simulink model "springdamper_model"  (R2020a)
settings: Solver=ode45  StartTime=0.0  StopTime=4  MaxStep=0.0009  MinStep=0.0001  RelTol=1e-3
values from neighbouring files (symbols this model uses):
  C_W = 1000    [springdamper_data.m]
  H_PC = 0.1265    [springdamper_data.m]
  H_RC_FRONT = 0.0346    [springdamper_data.m]
  H_RC_REAR = 0.0779    [springdamper_data.m]
  K_S = 26300    [springdamper_data.m]
  K_W = 50000    [springdamper_data.m]
  PC_TO_FRONT_AXLE = 0.667    [springdamper_data.m]
  PC_TO_REAR_AXLE = WHEELBASE-0.667    (= 0.873)    [springdamper_data.m]
  PITCH_INERTIA_PC = PITCH_INERTIA + SUSP_MASS*PC_TO_SUSPCOG^2    (= 73.7412)    [springdamper_data.m]
  pull = pull15431543    [springdamper_data.m]
  push = push15431543    [springdamper_data.m]
  QUARTER_MASS = 13    [springdamper_data.m]
  RC_TO_WHEEL_FRONT = TRACK_FRONT/2    (= 0.6)    [springdamper_data.m]
  RC_TO_WHEEL_REAR = TRACK_REAR/2    (= 0.58)    [springdamper_data.m]
  ROLL_INERTIA_RC = ROLL_INERTIA + SUSP_MASS*((RC_TO_SUSPCOG_FRONT+RC_TO_SUSPCOG_REAR)/2)^2    (= 22.694437)    [springdamper_data.m]
  SUSP_MASS = 208    [springdamper_data.m]
  SUSPCOG = 0.283    [springdamper_data.m]
  vel = [0 12.5 25 50 75 100 125 150 175 200 225 250]    [springdamper_data.m]
  WHEELBASE = 1.54    [springdamper_data.m]
  YAW_INERTIA = 63    [springdamper_data.m]
undefined symbols (not defined in the file or in its folder): sigbuilder_block
libraries: simulink_extras x6, simulink x3
(part 1 of 2)
settings Model: Creator=pungorpeter  LastModifiedBy=pungorpeter

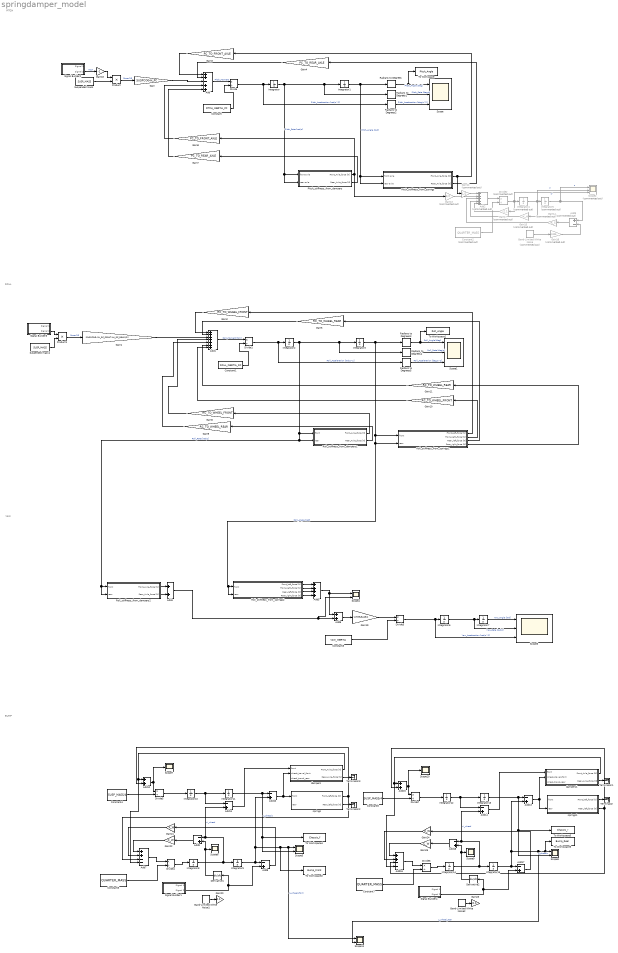
== system springdamper_model ==
  note: BUMP
  note: YAW
  note: ROLL
  note: PITCH
  Add : Sum  Inputs=++-++
  Add1 : Sum  Inputs=+++++++
  Add{8..11,13..14,17..18} (8 alike) : Sum  Inputs=-+
  Add{4,6,12,15} (4 alike) : Sum
  Add16 : Sum  Inputs=++--
  Add2 : Sum  Commented=on  Inputs=+++++
  Add3 : Sum  Commented=on  Inputs=+-
  Add5 : Sum  Inputs=++++
  Add7 : Sum  Inputs=++--
  Band-Limited White Noise : simulink/Sources/Band-Limited White Noise  Commented=on  Cov=[0.0005]  Ts=0.05  seed=[54341]
  Band-Limited White Noise1 : simulink/Sources/Band-Limited White Noise  Cov=[0.0005]  Ts=0.05  seed=[54341]
  Band-Limited White Noise2 : simulink/Sources/Band-Limited White Noise  Cov=[0.0005]  Ts=0.05  seed=[54341]
  Constant : Constant  Value=PITCH_INERTIA_PC
  Constant1 : Constant  Value=ROLL_INERTIA_RC
  Constant2 : Constant  Commented=on  Value=QUARTER_MASS
  Constant3 : Constant  Value=YAW_INERTIA
  Constant4 : Constant  Value=SUSP_MASS/4
  Constant5 : Constant  Value=QUARTER_MASS
  Constant6 : Constant  Value=SUSP_MASS/4
  Constant7 : Constant  Value=QUARTER_MASS
  Derivative1 : Derivative
  Derivative2 : Derivative
  Divide{,1,3..7} (7 alike) : Product  Inputs=*/
  Divide2 : Product  Commented=on  Inputs=*/
  Gain : Gain  Gain=SUSPCOG-H_PC
  Gain1 : Gain  Gain=(SUSPCOG-((H_RC_FRONT+H_RC_REAR)/2))
  Gain10 : Gain  Gain=RC_TO_WHEEL_FRONT
  Gain11 : Gain  Gain=RC_TO_WHEEL_REAR
  Gain12 : Gain  Commented=on  Gain=1/2
  Gain13 : Gain  Commented=on  Gain=1/2
  Gain14 : Gain  Commented=on  Gain=-K_S
  Gain15 : Gain  Commented=on  Gain=-K_W
  Gain16 : Gain  Commented=on  Gain=0.005
  Gain17 : Gain  Commented=on  Gain=-2.1
  Gain18 : Gain  Gain=-1
  Gain19 : Gain  Gain=WHEELBASE/2
  Gain2 : Gain  Gain=RC_TO_WHEEL_FRONT
  Gain20 : Gain  Gain=0.1
  Gain21 : Gain  Gain=K_W
  Gain22 : Gain  Gain=C_W
  Gain23 : Gain  Gain=0.1
  Gain24 : Gain  Gain=K_W
  Gain25 : Gain  Gain=C_W
  Gain3 : Gain  Gain=PC_TO_FRONT_AXLE
  Gain4 : Gain  Gain=PC_TO_REAR_AXLE
  Gain5 : Gain  Gain=RC_TO_WHEEL_REAR
  Gain6 : Gain  Gain=RC_TO_WHEEL_FRONT
  Gain7 : Gain  Gain=PC_TO_REAR_AXLE
  Gain8 : Gain  Gain=PC_TO_FRONT_AXLE
  Gain9 : Gain  Gain=RC_TO_WHEEL_REAR
  Integrator{,1..3,6..15} (14 alike) : Integrator
  Integrator4 : Integrator  Commented=on
  Integrator5 : Integrator  Commented=on
  Pitch_stiffness_from_dampers : Subsystem
  Pitch_stiffness_from_springs : Subsystem
  Product : Product
  Product1 : Product
  Radians to Degrees{,1..5} (6 alike) : simulink_extras/Transformations/Radians to Degrees
  Roll_stiffness_from_dampers1 : Subsystem
  Roll_stiffness_from_dampers2 : Subsystem
  Roll_stiffness_from_springs1 : Subsystem
  Roll_stiffness_from_springs2 : Subsystem
  Scope : Scope  NumInputPorts=3
  Scope1 : Scope  NumInputPorts=3
  Scope{6..7,9..10} (4 alike) : Scope
  Scope{4..5,8,11} (4 alike) : Scope  NumInputPorts=2
  Scope2 : Scope  Commented=on  NumInputPorts=3
  Scope3 : Scope  NumInputPorts=3
  Signal Builder1 : Subsystem  Tag=STV Subsys  LoadFcn=sigbuilder_block('load');  StartFcn=sigbuilder_block('start');  StopFcn=sigbuilder_block('stop');  ClipboardFcn=sigbuilder_block('clipboard');  mask(Sigbuilder block){tuvar=[0:10]}
      mask help: Simulink:masks:SigbuilderBlock_MD
      mask init:
      | if ~strcmp(get_param(bdroot(gcbh),'SimulationStatus'),'stopped') tuvar = sigbuilder_block('maskInit'); end
      settings: CopyFcn=sigbuilder_block('copy');  DeleteFcn=sigbuilder_block('delete');  ModelCloseFcn=sigbuilder_block('modelClose');  PreSaveFcn=sigbuilder_block('preSave');  PauseFcn=sigbuilder_block('pause');  ContinueFcn=sigbuilder_block('continue');  NameChangeFcn=sigbuilder_block('namechange');  OpenFcn=sigbuilder_block('open',[346.8 134.4 550.8 400.2 ]);  CloseFcn=sigbuilder_block('close');
      mask Display: plot(0, 0, 100, 100,[2, 2, 32, 32, 2], [68, 8, 8, 68, 68],[32, 2], [38, 38], [32, 19, 2],[53, 60, 44], [32, 17, 17, 2],[16, 16, 31, 31]);txt = getActiveGroup(gcbh);text(2, 100, txt,'verticalAlignment', 'top');
  Signal Builder2 : Subsystem  Tag=STV Subsys  LoadFcn=sigbuilder_block('load');  StartFcn=sigbuilder_block('start');  StopFcn=sigbuilder_block('stop');  ClipboardFcn=sigbuilder_block('clipboard');  mask(Sigbuilder block){tuvar=[0:10]}
      mask help: Simulink:masks:SigbuilderBlock_MD
      mask init:
      | if ~strcmp(get_param(bdroot(gcbh),'SimulationStatus'),'stopped') tuvar = sigbuilder_block('maskInit'); end
      settings: CopyFcn=sigbuilder_block('copy');  DeleteFcn=sigbuilder_block('delete');  ModelCloseFcn=sigbuilder_block('modelClose');  PreSaveFcn=sigbuilder_block('preSave');  PauseFcn=sigbuilder_block('pause');  ContinueFcn=sigbuilder_block('continue');  NameChangeFcn=sigbuilder_block('namechange');  OpenFcn=sigbuilder_block('open',[346.8 134.4 550.8 400.2 ]);  CloseFcn=sigbuilder_block('close');
      mask Display: plot(0, 0, 100, 100,[2, 2, 32, 32, 2], [68, 8, 8, 68, 68],[32, 2], [38, 38], [32, 19, 2],[53, 60, 44], [32, 17, 17, 2],[16, 16, 31, 31]);txt = getActiveGroup(gcbh);text(2, 100, txt,'verticalAlignment', 'top');
  Signal Builder3 : Subsystem  Tag=STV Subsys  LoadFcn=sigbuilder_block('load');  StartFcn=sigbuilder_block('start');  StopFcn=sigbuilder_block('stop');  ClipboardFcn=sigbuilder_block('clipboard');  mask(Sigbuilder block){tuvar=[0:10]}
      mask help: Simulink:masks:SigbuilderBlock_MD
      mask init:
      | if ~strcmp(get_param(bdroot(gcbh),'SimulationStatus'),'stopped') tuvar = sigbuilder_block('maskInit'); end
      settings: CopyFcn=sigbuilder_block('copy');  DeleteFcn=sigbuilder_block('delete');  ModelCloseFcn=sigbuilder_block('modelClose');  PreSaveFcn=sigbuilder_block('preSave');  PauseFcn=sigbuilder_block('pause');  ContinueFcn=sigbuilder_block('continue');  NameChangeFcn=sigbuilder_block('namechange');  OpenFcn=sigbuilder_block('open',[346.8 134.4 550.8 400.2 ]);  CloseFcn=sigbuilder_block('close');
      mask Display: plot(0, 0, 100, 100,[2, 2, 32, 32, 2], [68, 8, 8, 68, 68],[32, 2], [38, 38], [32, 19, 2],[53, 60, 44], [32, 17, 17, 2],[16, 16, 31, 31]);txt = getActiveGroup(gcbh);text(2, 100, txt,'verticalAlignment', 'top');
  Signal Builder4 : Subsystem  Tag=STV Subsys  LoadFcn=sigbuilder_block('load');  StartFcn=sigbuilder_block('start');  StopFcn=sigbuilder_block('stop');  ClipboardFcn=sigbuilder_block('clipboard');  mask(Sigbuilder block){tuvar=[0:10]}
      mask help: Simulink:masks:SigbuilderBlock_MD
      mask init:
      | if ~strcmp(get_param(bdroot(gcbh),'SimulationStatus'),'stopped') tuvar = sigbuilder_block('maskInit'); end
      settings: CopyFcn=sigbuilder_block('copy');  DeleteFcn=sigbuilder_block('delete');  ModelCloseFcn=sigbuilder_block('modelClose');  PreSaveFcn=sigbuilder_block('preSave');  PauseFcn=sigbuilder_block('pause');  ContinueFcn=sigbuilder_block('continue');  NameChangeFcn=sigbuilder_block('namechange');  OpenFcn=sigbuilder_block('open',[346.8 134.4 550.8 400.2 ]);  CloseFcn=sigbuilder_block('close');
      mask Display: plot(0, 0, 100, 100,[2, 2, 32, 32, 2], [68, 8, 8, 68, 68],[32, 2], [38, 38], [32, 19, 2],[53, 60, 44], [32, 17, 17, 2],[16, 16, 31, 31]);txt = getActiveGroup(gcbh);text(2, 100, txt,'verticalAlignment', 'top');
  Suspended mass : Constant  Value=SUSP_MASS
  Suspended mass1 : Constant  Value=SUSP_MASS
  Terminator{,1..3} (4 alike) : Terminator
  To Workspace : ToWorkspace  VariableName=Pitch_Angle  SampleTime=-1
  To Workspace1 : ToWorkspace  VariableName=Roll_Angle  SampleTime=-1
  To Workspace2 : ToWorkspace  VariableName=Bump_Front  SampleTime=-1
  To Workspace3 : ToWorkspace  VariableName=Bump_Rear  SampleTime=-1
  To Workspace4 : ToWorkspace  VariableName=Chassis_f  SampleTime=-1
  To Workspace5 : ToWorkspace  VariableName=Chassis_r  SampleTime=-1
  dampers : Subsystem
  dampers1 : Subsystem
  springs : Subsystem
  springs1 : Subsystem
  wires:
  Signal Builder2/2(Signal 2) -> Gain18/1  "AccX"
  Suspended mass/1 -> Product/2
  Product/1 -> Gain/1  "Force [N]"
  Gain/1 -> Add/3
  Divide/1 -> Radians to Degrees2/1, Integrator/1  "Pitch_Acceleration [rad/s^2]"
  Integrator/1 -> Radians to Degrees1/1, Integrator1/1, Pitch_stiffness_from_dampers/2("rear axle "), Pitch_stiffness_from_dampers/1("front axle ")  "Pitch_Rate [rad/s]"
  Constant/1 -> Divide/2
  Integrator1/1 -> Pitch_stiffness_from_springs/2(rear axle), Pitch_stiffness_from_springs/1(front axle), Radians to Degrees/1  "Pitch_Angle [rad]"
  Add/1 -> Divide/1  "Pitch_Moment"
  Gain3/1 -> Add/1
  Gain4/1 -> Add/2
  Radians to Degrees/1 -> To Workspace/1, Scope/1  "Pitch_Angle [deg]"
  Pitch_stiffness_from_springs/1(Front_Axle_force [N]) -> Gain3/1, Gain12/1
  Pitch_stiffness_from_springs/2(Rear_Axle_force [N]) -> Gain4/1
  Gain8/1 -> Add/4
  Gain7/1 -> Add/5
  Radians to Degrees1/1 -> Scope/2  "Pitch_Rate [deg/s]"
  Radians to Degrees2/1 -> Scope/3  "Pitch_Acceleration [deg/s^2]"
  Pitch_stiffness_from_dampers/2(Rear_Axle_force [N]) -> Gain7/1
  Pitch_stiffness_from_dampers/1(Front_Axle_force [N]) -> Gain13/1, Gain8/1
  Gain9/1 -> Add1/5
  Gain2/1 -> Add1/1
  Roll_stiffness_from_dampers1/1(Front_Axle_force [N]) -> Gain6/1
  Roll_stiffness_from_dampers1/2(Rear_Axle_force [N]) -> Gain9/1
  Divide1/1 -> Radians to Degrees5/1, Integrator2/1  "Roll_Acceleration [rad/s^2]"
  Radians to Degrees4/1 -> Scope1/2  "Roll_Rate [deg/s]"
  Integrator3/1 -> Roll_stiffness_from_springs2/2(rear), Roll_stiffness_from_springs2/1(front), Roll_stiffness_from_springs1/2(rear), Roll_stiffness_from_springs1/1(front), Radians to Degrees3/1  "Roll_Angle [rad]"
  Gain5/1 -> Add1/2
  Gain6/1 -> Add1/4
  Roll_stiffness_from_springs1/3(Rear_left_force [N]) -> Gain5/1
  Radians to Degrees3/1 -> To Workspace1/1, Scope1/1  "Roll_Angle [deg]"
  Add1/1 -> Divide1/1  "Roll_Moment [Nm]"
  Integrator2/1 -> Radians to Degrees4/1, Integrator3/1, Roll_stiffness_from_dampers2/2("rear "), Roll_stiffness_from_dampers2/1("front "), Roll_stiffness_from_dampers1/2("rear "), Roll_stiffness_from_dampers1/1("front ")  "Roll_Rate [rad/s]"
  Constant1/1 -> Divide1/2
  Product1/1 -> Gain1/1  "Force [N]"
  Signal Builder3/2(Signal 2) -> Product1/1
  Suspended mass1/1 -> Product1/2
  Gain1/1 -> Add1/3
  Radians to Degrees5/1 -> Scope1/3  "Roll_Acceleration [deg/s^2]"
  Roll_stiffness_from_springs1/1(Front_left_force [N]) -> Gain2/1
  Roll_stiffness_from_springs1/2(Front_right_force [N]) -> Gain10/1
  Roll_stiffness_from_springs1/4(Rear_right_force [N]) -> Gain11/1
  Gain11/1 -> Add1/6
  Gain10/1 -> Add1/7
  Gain12/1 -> Add2/1
  Constant2/1 -> Divide2/2
  Divide2/1 -> Gain17/1, Scope2/3, Integrator4/1  "z''"
  Integrator4/1 -> Gain15/1, Scope2/2, Integrator5/1  "z'"
  Integrator5/1 -> Add3/1, Scope2/1  "z"
  Gain13/1 -> Add2/2
  Add2/1 -> Divide2/1
  Gain14/1 -> Add2/3
  Gain15/1 -> Add2/4
  Band-Limited White Noise/1 -> Gain16/1
  Gain16/1 -> Add3/2
  Gain17/1 -> Add2/5
  Add3/1 -> Gain14/1
  Gain18/1 -> Product/1
  Constant3/1 -> Divide3/2
  Roll_stiffness_from_dampers2/1(Front_Axle_force [N]) -> Add4/1
  Roll_stiffness_from_dampers2/2(Rear_Axle_force [N]) -> Add4/2
  Roll_stiffness_from_springs2/1(Front_left_force [N]) -> Add5/1
  Roll_stiffness_from_springs2/2(Front_right_force [N]) -> Add5/2
  Roll_stiffness_from_springs2/3(Rear_left_force [N]) -> Add5/3
  Roll_stiffness_from_springs2/4(Rear_right_force [N]) -> Add5/4
  Add4/1 -> Scope4/2, Add6/2
  Add5/1 -> Add6/1, Scope4/1
  Add6/1 -> Gain19/1
  Gain19/1 -> Divide3/1
  Divide3/1 -> Scope3/3, Integrator6/1  "Yaw_Acceleration [rad/s^2]"
  Integrator6/1 -> Scope3/2, Integrator7/1  "Yaw_Rate [rad/s]"
  Integrator7/1 -> Scope3/1  "Yaw_Angle [rad]"
  Constant5/1 -> Divide4/2
  Divide4/1 -> Integrator8/1
  Integrator8/1 -> Integrator9/1, Add11/2, Add9/1  "z'_wheel"
  Integrator10/1 -> Integrator11/1, Add11/1
  Divide5/1 -> Integrator10/1
  Constant4/1 -> Divide5/2
  Gain22/1 -> Add7/1
  Add7/1 -> Divide4/1
  Gain21/1 -> Add7/2
  Add8/1 -> Gain21/1
  Integrator11/1 -> Scope5/2, To Workspace4/1, Add10/1  "z_chassis"
  Integrator9/1 -> To Workspace2/1, Scope11/1, Scope5/1, Add10/2, Add8/1  "z_wheel_front"
  Band-Limited White Noise1/1 -> Gain20/1
  Add9/1 -> Gain22/1
  Derivative1/1 -> Scope6/1, Add9/2
  springs/1(Front_left_force [N]) -> Add7/3, Add12/2
  Add10/1 -> dampers/2(wheek_travel_front), springs/1(front)
  Add12/1 -> Divide5/1, Scope7/1
  Add11/1 -> dampers/1("front ")
  dampers/1(Front_Axle_force [N]) -> Add7/4, Add12/1
  Signal Builder1/2(Signal 2) -> Add8/2, Derivative1/1
  Band-Limited White Noise2/1 -> Gain23/1
  Add17/1 -> Gain24/1
  Add15/1 -> Divide7/1, Scope10/1
  Integrator12/1 -> Integrator13/1, Add14/1
  Add18/1 -> Gain25/1
  Add14/1 -> dampers1/1("front ")
  Add13/1 -> springs1/2(rear), dampers1/2(wheek_travel_front)
  dampers1/1(Front_Axle_force [N]) -> Add16/4, Add15/1
  Derivative2/1 -> Scope9/1, Add18/2
  Divide6/1 -> Integrator14/1
  Integrator14/1 -> Integrator15/1, Add14/2, Add18/1  "z'_wheel"
  Add16/1 -> Divide6/1
  Signal Builder4/2(Signal 2) -> Add17/2, Derivative2/1
  Integrator15/1 -> Scope11/2, To Workspace3/1, Scope8/1, Add13/2, Add17/1  "z_wheel_rear"
  Constant7/1 -> Divide6/2
  Constant6/1 -> Divide7/2
  Gain24/1 -> Add16/2
  Gain25/1 -> Add16/1
  Integrator13/1 -> To Workspace5/1, Scope8/2, Add13/1  "z_chassis"
  Divide7/1 -> Integrator12/1
  springs1/2(Rear_left_force [N]) -> Add16/3, Add15/2
  springs1/1(Front_left_force [N]) -> Terminator/1
  dampers1/2(Rear_Axle_force [N]) -> Terminator1/1
  springs/2(Rear_left_force [N]) -> Terminator2/1
  dampers/2(Rear_Axle_force [N]) -> Terminator3/1

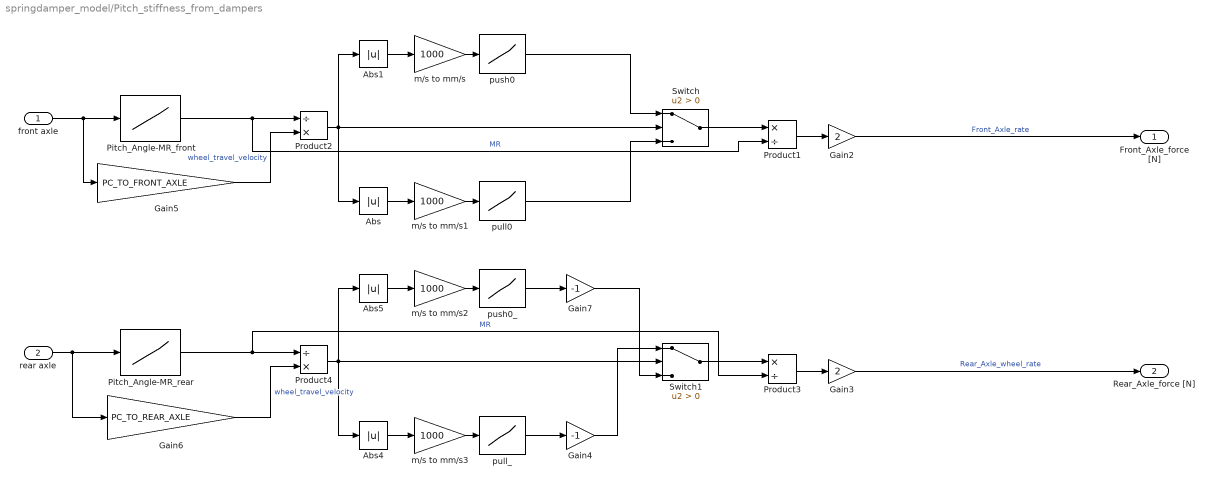
== system springdamper_model/Pitch_stiffness_from_dampers ==
  "front axle " : Inport
  "rear axle " : Inport  Port=2
  Abs{,1,4..5} (4 alike) : Abs
  Gain2 : Gain  Gain=2
  Gain3 : Gain  Gain=2
  Gain4 : Gain  Gain=-1
  Gain5 : Gain  Gain=PC_TO_FRONT_AXLE
  Gain6 : Gain  Gain=PC_TO_REAR_AXLE
  Gain7 : Gain  Gain=-1
  Pitch_Angle-MR_front : Lookup_n-D  NumberOfTableDimensions=1  BreakpointsForDimension1=[-0.026179939 -0.023561945 -0.020943951 -0.018325957 -0.015707963 -0.013089969 -0.010471976 -0.007853982 -0.005235988 -0.002617994 0 0.002617994 0.005235988 0.007853982 0.010471976 0.013089969 0.015707963 0.018325957 0.020943951 0.023561945 0.026179939]  Table=[1.257198381 1.24219912 1.227378639 1.212724626 1.198231914 1.183896009 1.169713083 1.155679982 1.141794232 1.128054061 1.114458431 1.10100708 1.087700579 1.074540406 1.061529036 1.048670055 1.035968301 1.023430037 1.011063164 0.998877485 0.986885031]  InternalRulePriority=Speed  RndMeth=Simplest  InputSameDT=on
  Pitch_Angle-MR_rear : Lookup_n-D  NumberOfTableDimensions=1  BreakpointsForDimension1=[-0.026179939 -0.023561945 -0.020943951 -0.018325957 -0.015707963 -0.013089969 -0.010471976 -0.007853982 -0.005235988 -0.002617994 0 0.002617994 0.005235988 0.007853982 0.010471976 0.013089969 0.015707963 0.018325957 0.020943951 0.023561945 0.026179939]  Table=[0.920766238 0.93127438 0.94215653 0.953367022 0.964872809 0.976646487 0.988665288 1.000910292 1.01336579 1.026018792 1.038858614 1.051876555 1.065065629 1.07842035 1.091936553 1.105611246 1.119442496 1.133429327 1.147571642 1.16187016 1.176326364]  InternalRulePriority=Speed  RndMeth=Simplest  InputSameDT=on
  Product1 : Product  Inputs=*/
  Product2 : Product  Inputs=/*
  Product3 : Product  Inputs=*/
  Product4 : Product  Inputs=/*
  Switch : Switch  Criteria=u2 > Threshold
  Switch1 : Switch  Criteria=u2 > Threshold
  m/s to mm/s{,1..3} (4 alike) : Gain  Gain=1000
  pull0 : Lookup_n-D  NumberOfTableDimensions=1  BreakpointsForDimension1=vel  Table=pull  InternalRulePriority=Speed  RndMeth=Simplest  InputSameDT=on
  pull_ : Lookup_n-D  NumberOfTableDimensions=1  BreakpointsForDimension1=vel  Table=pull  InternalRulePriority=Speed  RndMeth=Simplest  InputSameDT=on
  push0 : Lookup_n-D  NumberOfTableDimensions=1  BreakpointsForDimension1=vel  Table=push  InternalRulePriority=Speed  RndMeth=Simplest  InputSameDT=on
  push0_ : Lookup_n-D  NumberOfTableDimensions=1  BreakpointsForDimension1=vel  Table=push  InternalRulePriority=Speed  RndMeth=Simplest  InputSameDT=on
  Front_Axle_force [N] : Outport
  Rear_Axle_force [N] : Outport  Port=2
  wires:
  Gain2/1 -> Front_Axle_force [N]/1  "Front_Axle_rate"
  Gain3/1 -> Rear_Axle_force [N]/1  "Rear_Axle_wheel_rate"
  Pitch_Angle-MR_front/1 -> Product1/2, Product2/1  "MR"
  "front axle "/1 -> Gain5/1, Pitch_Angle-MR_front/1
  "rear axle "/1 -> Gain6/1, Pitch_Angle-MR_rear/1
  Gain5/1 -> Product2/2  "wheel_travel_velocity"
  Product2/1 -> Abs/1, Abs1/1, Switch/2
  m/s to mm/s/1 -> push0/1
  m/s to mm/s1/1 -> pull0/1
  Abs/1 -> m/s to mm/s1/1
  Abs1/1 -> m/s to mm/s/1
  Switch/1 -> Product1/1
  Product1/1 -> Gain2/1
  push0/1 -> Switch/1
  pull0/1 -> Switch/3
  push0_/1 -> Gain7/1
  m/s to mm/s3/1 -> pull_/1
  m/s to mm/s2/1 -> push0_/1
  Product4/1 -> Abs4/1, Abs5/1, Switch1/2
  Pitch_Angle-MR_rear/1 -> Product3/2, Product4/1  "MR"
  Switch1/1 -> Product3/1
  Abs4/1 -> m/s to mm/s3/1
  Gain6/1 -> Product4/2  "wheel_travel_velocity"
  Abs5/1 -> m/s to mm/s2/1
  Product3/1 -> Gain3/1
  pull_/1 -> Gain4/1
  Gain4/1 -> Switch1/1
  Gain7/1 -> Switch1/3

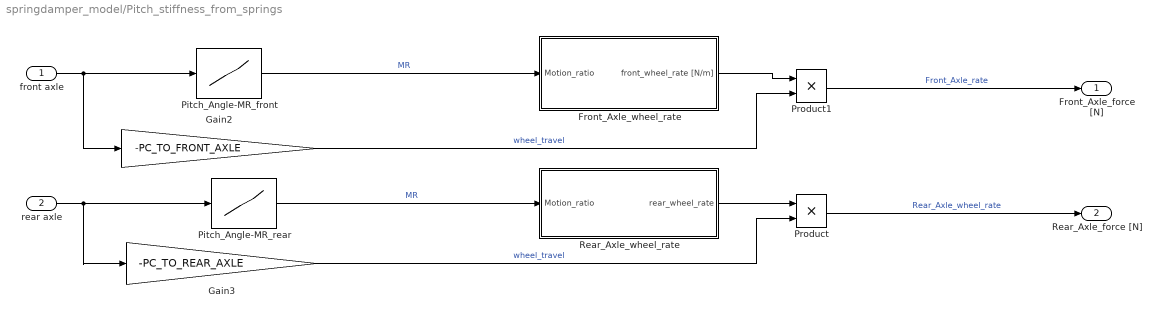
== system springdamper_model/Pitch_stiffness_from_springs ==
  front axle : Inport
  rear axle : Inport  Port=2
  Front_Axle_wheel_rate : Subsystem
  Gain2 : Gain  Gain=-PC_TO_FRONT_AXLE
  Gain3 : Gain  Gain=-PC_TO_REAR_AXLE
  Pitch_Angle-MR_front : Lookup_n-D  NumberOfTableDimensions=1  BreakpointsForDimension1=[-0.026179939 -0.023561945 -0.020943951 -0.018325957 -0.015707963 -0.013089969 -0.010471976 -0.007853982 -0.005235988 -0.002617994 0 0.002617994 0.005235988 0.007853982 0.010471976 0.013089969 0.015707963 0.018325957 0.020943951 0.023561945 0.026179939]  Table=[1.257198381 1.24219912 1.227378639 1.212724626 1.198231914 1.183896009 1.169713083 1.155679982 1.141794232 1.128054061 1.114458431 1.10100708 1.087700579 1.074540406 1.061529036 1.048670055 1.035968301 1.023430037 1.011063164 0.998877485 0.986885031]  InternalRulePriority=Speed  RndMeth=Simplest  InputSameDT=on
  Pitch_Angle-MR_rear : Lookup_n-D  NumberOfTableDimensions=1  BreakpointsForDimension1=[-0.026179939 -0.023561945 -0.020943951 -0.018325957 -0.015707963 -0.013089969 -0.010471976 -0.007853982 -0.005235988 -0.002617994 0 0.002617994 0.005235988 0.007853982 0.010471976 0.013089969 0.015707963 0.018325957 0.020943951 0.023561945 0.026179939]  Table=[0.920766238 0.93127438 0.94215653 0.953367022 0.964872809 0.976646487 0.988665288 1.000910292 1.01336579 1.026018792 1.038858614 1.051876555 1.065065629 1.07842035 1.091936553 1.105611246 1.119442496 1.133429327 1.147571642 1.16187016 1.176326364]  InternalRulePriority=Speed  RndMeth=Simplest  InputSameDT=on
  Product : Product
  Product1 : Product
  Rear_Axle_wheel_rate : Subsystem
  Front_Axle_force [N] : Outport
  Rear_Axle_force [N] : Outport  Port=2
  wires:
  Front_Axle_wheel_rate/1(front_wheel_rate [N/m]) -> Product1/1
  Product1/1 -> Front_Axle_force [N]/1  "Front_Axle_rate"
  Product/1 -> Rear_Axle_force [N]/1  "Rear_Axle_wheel_rate"
  front axle/1 -> Gain2/1, Pitch_Angle-MR_front/1
  rear axle/1 -> Pitch_Angle-MR_rear/1, Gain3/1
  Gain2/1 -> Product1/2  "wheel_travel"
  Gain3/1 -> Product/2  "wheel_travel"
  Pitch_Angle-MR_rear/1 -> Rear_Axle_wheel_rate/1(Motion_ratio)  "MR"
  Pitch_Angle-MR_front/1 -> Front_Axle_wheel_rate/1(Motion_ratio)  "MR"
  Rear_Axle_wheel_rate/1(rear_wheel_rate) -> Product/1

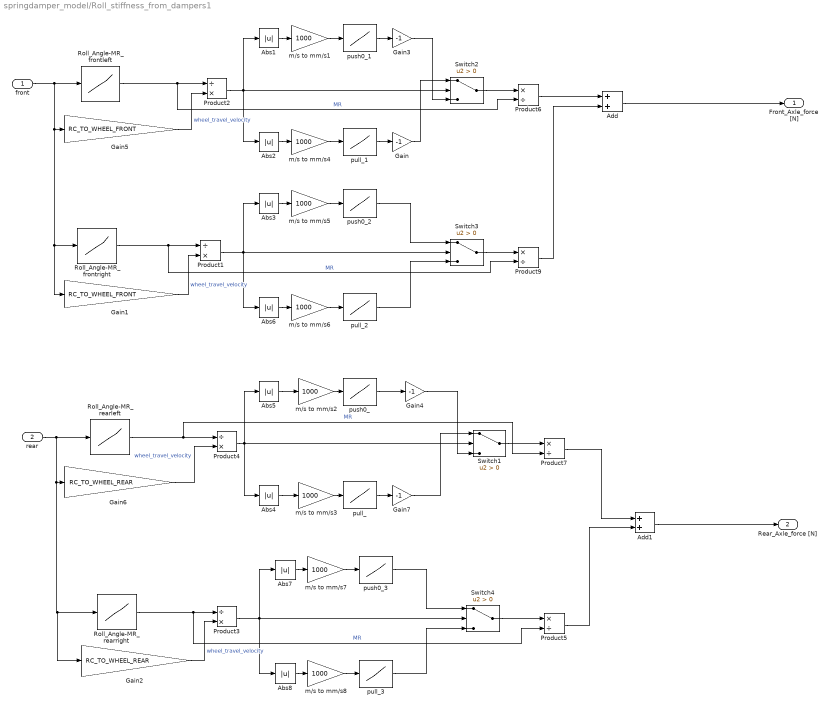
== system springdamper_model/Roll_stiffness_from_dampers1 ==
  "front " : Inport
  "rear " : Inport  Port=2
  Abs{1..8} (8 alike) : Abs
  Add : Sum
  Add1 : Sum
  Gain{,3..4,7} (4 alike) : Gain  Gain=-1
  Gain1 : Gain  Gain=RC_TO_WHEEL_FRONT
  Gain2 : Gain  Gain=RC_TO_WHEEL_REAR
  Gain5 : Gain  Gain=RC_TO_WHEEL_FRONT
  Gain6 : Gain  Gain=RC_TO_WHEEL_REAR
  Product{1..4} (4 alike) : Product  Inputs=/*
  Product{5..7,9} (4 alike) : Product  Inputs=*/
  Roll_Angle-MR_frontleft : Lookup_n-D  NumberOfTableDimensions=1  BreakpointsForDimension1=[-0.02618 -0.02356 -0.02094 -0.01833 -0.01571 -0.01309 -0.01047 -0.00785 -0.00524 -0.00262 0.00000 0.00262 0.00524 0.00785 0.01047 0.01309 0.01571 0.01833 0.02094 0.02356 0.02618]  Table=[1.013 1.023 1.032 1.042 1.052 1.062 1.073 1.083 1.093 1.104 1.114 1.125 1.136 1.147 1.158 1.169 1.181 1.192 1.204 1.215 1.227]  InternalRulePriority=Speed  RndMeth=Simplest  InputSameDT=on
  Roll_Angle-MR_frontright : Lookup_n-D  NumberOfTableDimensions=1  BreakpointsForDimension1=[-0.02618 -0.02356 -0.02094 -0.01833 -0.01571 -0.01309 -0.01047 -0.00785 -0.00524 -0.00262 0.00000 0.00262 0.00524 0.00785 0.01047 0.01309 0.01571 0.01833 0.02094 0.02356 0.02618]  Table=[1.227 1.215 1.204 1.192 1.181 1.169 1.158 1.147 1.136 1.125 1.115 1.104 1.093 1.083 1.073 1.062 1.052 1.042 1.032 1.023 1.013]  InternalRulePriority=Speed  RndMeth=Simplest  InputSameDT=on
  Roll_Angle-MR_rearleft : Lookup_n-D  NumberOfTableDimensions=1  BreakpointsForDimension1=[-0.02618 -0.02356 -0.02094 -0.01833 -0.01571 -0.01309 -0.01047 -0.00785 -0.00524 -0.00262 0.00000 0.00262 0.00524 0.00785 0.01047 0.01309 0.01571 0.01833 0.02094 0.02356 0.02618]  Table=[0.945 0.953 0.962 0.971 0.980 0.990 0.999 1.009 1.019 1.029 1.039 1.049 1.059 1.070 1.080 1.091 1.102 1.113 1.124 1.135 1.147]  InternalRulePriority=Speed  RndMeth=Simplest  InputSameDT=on
  Roll_Angle-MR_rearright : Lookup_n-D  NumberOfTableDimensions=1  BreakpointsForDimension1=[-0.02618 -0.02356 -0.02094 -0.01833 -0.01571 -0.01309 -0.01047 -0.00785 -0.00524 -0.00262 0.00000 0.00262 0.00524 0.00785 0.01047 0.01309 0.01571 0.01833 0.02094 0.02356 0.02618]  Table=[1.147 1.135 1.124 1.113 1.102 1.091 1.080 1.070 1.059 1.049 1.039 1.029 1.019 1.009 0.999 0.990 0.980 0.971 0.962 0.953 0.945]  InternalRulePriority=Speed  RndMeth=Simplest  InputSameDT=on
  Switch{1..4} (4 alike) : Switch  Criteria=u2 > Threshold
  m/s to mm/s{1..8} (8 alike) : Gain  Gain=1000
  pull_{,1..3} (4 alike) : Lookup_n-D  NumberOfTableDimensions=1  BreakpointsForDimension1=vel  Table=pull  InternalRulePriority=Speed  RndMeth=Simplest  InputSameDT=on
  push0_{,1..3} (4 alike) : Lookup_n-D  NumberOfTableDimensions=1  BreakpointsForDimension1=vel  Table=push  InternalRulePriority=Speed  RndMeth=Simplest  InputSameDT=on
  Front_Axle_force [N] : Outport
  Rear_Axle_force [N] : Outport  Port=2
  wires:
  Switch2/1 -> Product6/1
  Add1/1 -> Rear_Axle_force [N]/1
  Roll_Angle-MR_frontleft/1 -> Product6/2, Product2/1  "MR"
  "front "/1 -> Roll_Angle-MR_frontleft/1, Gain1/1, Roll_Angle-MR_frontright/1, Gain5/1
  "rear "/1 -> Roll_Angle-MR_rearleft/1, Gain2/1, Roll_Angle-MR_rearright/1, Gain6/1
  Gain5/1 -> Product2/2  "wheel_travel_velocity"
  m/s to mm/s3/1 -> pull_/1
  m/s to mm/s2/1 -> push0_/1
  Product4/1 -> Abs4/1, Abs5/1, Switch1/2
  Roll_Angle-MR_rearleft/1 -> Product7/2, Product4/1  "MR"
  Switch1/1 -> Product7/1
  Abs4/1 -> m/s to mm/s3/1
  Gain6/1 -> Product4/2  "wheel_travel_velocity"
  Abs5/1 -> m/s to mm/s2/1
  Product7/1 -> Add1/1
  pull_/1 -> Gain7/1
  push0_/1 -> Gain4/1
  Abs1/1 -> m/s to mm/s1/1
  Product2/1 -> Abs2/1, Switch2/2, Abs1/1
  m/s to mm/s1/1 -> push0_1/1
  pull_1/1 -> Gain/1
  Abs2/1 -> m/s to mm/s4/1
  m/s to mm/s4/1 -> pull_1/1
  push0_1/1 -> Gain3/1
  Roll_Angle-MR_frontright/1 -> Product9/2, Product1/1  "MR"
  Gain1/1 -> Product1/2  "wheel_travel_velocity"
  push0_2/1 -> Switch3/1
  m/s to mm/s6/1 -> pull_2/1
  Abs6/1 -> m/s to mm/s6/1
  m/s to mm/s5/1 -> push0_2/1
  Product1/1 -> Abs6/1, Abs3/1, Switch3/2
  Abs3/1 -> m/s to mm/s5/1
  pull_2/1 -> Switch3/3
  Product9/1 -> Add/2
  Add/1 -> Front_Axle_force [N]/1
  push0_3/1 -> Switch4/1
  Product5/1 -> Add1/2
  Abs7/1 -> m/s to mm/s7/1
  Gain2/1 -> Product3/2  "wheel_travel_velocity"
  m/s to mm/s8/1 -> pull_3/1
  pull_3/1 -> Switch4/3
  m/s to mm/s7/1 -> push0_3/1
  Product3/1 -> Abs8/1, Abs7/1, Switch4/2
  Abs8/1 -> m/s to mm/s8/1
  Roll_Angle-MR_rearright/1 -> Product5/2, Product3/1  "MR"
  Product6/1 -> Add/1
  Switch3/1 -> Product9/1
  Switch4/1 -> Product5/1
  Gain/1 -> Switch2/1
  Gain3/1 -> Switch2/3
  Gain4/1 -> Switch1/3
  Gain7/1 -> Switch1/1

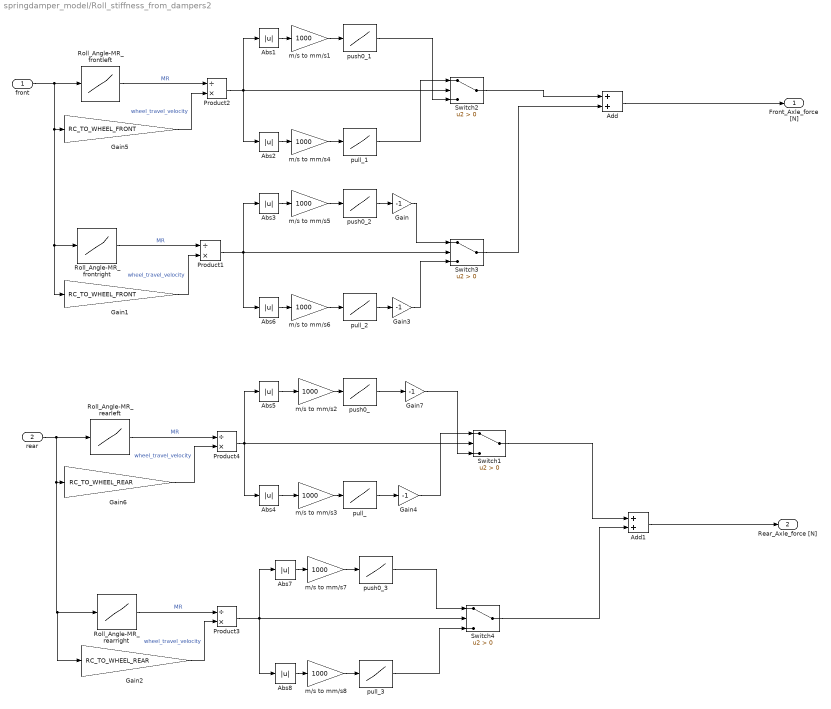
== system springdamper_model/Roll_stiffness_from_dampers2 ==
  "front " : Inport
  "rear " : Inport  Port=2
  Abs{1..8} (8 alike) : Abs
  Add : Sum
  Add1 : Sum
  Gain{,3..4,7} (4 alike) : Gain  Gain=-1
  Gain1 : Gain  Gain=RC_TO_WHEEL_FRONT
  Gain2 : Gain  Gain=RC_TO_WHEEL_REAR
  Gain5 : Gain  Gain=RC_TO_WHEEL_FRONT
  Gain6 : Gain  Gain=RC_TO_WHEEL_REAR
  Product{1..4} (4 alike) : Product  Inputs=/*
  Roll_Angle-MR_frontleft : Lookup_n-D  NumberOfTableDimensions=1  BreakpointsForDimension1=[-0.02618 -0.02356 -0.02094 -0.01833 -0.01571 -0.01309 -0.01047 -0.00785 -0.00524 -0.00262 0.00000 0.00262 0.00524 0.00785 0.01047 0.01309 0.01571 0.01833 0.02094 0.02356 0.02618]  Table=[1.013 1.023 1.032 1.042 1.052 1.062 1.073 1.083 1.093 1.104 1.114 1.125 1.136 1.147 1.158 1.169 1.181 1.192 1.204 1.215 1.227]  InternalRulePriority=Speed  RndMeth=Simplest  InputSameDT=on
  Roll_Angle-MR_frontright : Lookup_n-D  NumberOfTableDimensions=1  BreakpointsForDimension1=[-0.02618 -0.02356 -0.02094 -0.01833 -0.01571 -0.01309 -0.01047 -0.00785 -0.00524 -0.00262 0.00000 0.00262 0.00524 0.00785 0.01047 0.01309 0.01571 0.01833 0.02094 0.02356 0.02618]  Table=[1.227 1.215 1.204 1.192 1.181 1.169 1.158 1.147 1.136 1.125 1.115 1.104 1.093 1.083 1.073 1.062 1.052 1.042 1.032 1.023 1.013]  InternalRulePriority=Speed  RndMeth=Simplest  InputSameDT=on
  Roll_Angle-MR_rearleft : Lookup_n-D  NumberOfTableDimensions=1  BreakpointsForDimension1=[-0.02618 -0.02356 -0.02094 -0.01833 -0.01571 -0.01309 -0.01047 -0.00785 -0.00524 -0.00262 0.00000 0.00262 0.00524 0.00785 0.01047 0.01309 0.01571 0.01833 0.02094 0.02356 0.02618]  Table=[0.945 0.953 0.962 0.971 0.980 0.990 0.999 1.009 1.019 1.029 1.039 1.049 1.059 1.070 1.080 1.091 1.102 1.113 1.124 1.135 1.147]  InternalRulePriority=Speed  RndMeth=Simplest  InputSameDT=on
  Roll_Angle-MR_rearright : Lookup_n-D  NumberOfTableDimensions=1  BreakpointsForDimension1=[-0.02618 -0.02356 -0.02094 -0.01833 -0.01571 -0.01309 -0.01047 -0.00785 -0.00524 -0.00262 0.00000 0.00262 0.00524 0.00785 0.01047 0.01309 0.01571 0.01833 0.02094 0.02356 0.02618]  Table=[1.147 1.135 1.124 1.113 1.102 1.091 1.080 1.070 1.059 1.049 1.039 1.029 1.019 1.009 0.999 0.990 0.980 0.971 0.962 0.953 0.945]  InternalRulePriority=Speed  RndMeth=Simplest  InputSameDT=on
  Switch{1..4} (4 alike) : Switch  Criteria=u2 > Threshold
  m/s to mm/s{1..8} (8 alike) : Gain  Gain=1000
  pull_{,1..3} (4 alike) : Lookup_n-D  NumberOfTableDimensions=1  BreakpointsForDimension1=vel  Table=pull  InternalRulePriority=Speed  RndMeth=Simplest  InputSameDT=on
  push0_{,1..3} (4 alike) : Lookup_n-D  NumberOfTableDimensions=1  BreakpointsForDimension1=vel  Table=push  InternalRulePriority=Speed  RndMeth=Simplest  InputSameDT=on
  Front_Axle_force [N] : Outport
  Rear_Axle_force [N] : Outport  Port=2
  wires:
  pull_/1 -> Gain4/1
  push0_/1 -> Gain7/1
  push0_1/1 -> Switch2/3
  pull_1/1 -> Switch2/1
  Switch2/1 -> Add/1
  Roll_Angle-MR_rearright/1 -> Product3/1  "MR"
  Abs8/1 -> m/s to mm/s8/1
  Product3/1 -> Switch4/2, Abs7/1, Abs8/1
  m/s to mm/s7/1 -> push0_3/1
  pull_3/1 -> Switch4/3
  m/s to mm/s8/1 -> pull_3/1
  Gain2/1 -> Product3/2  "wheel_travel_velocity"
  Abs7/1 -> m/s to mm/s7/1
  Switch4/1 -> Add1/2
  Add/1 -> Front_Axle_force [N]/1
  Switch3/1 -> Add/2
  pull_2/1 -> Gain3/1
  Abs3/1 -> m/s to mm/s5/1
  Product1/1 -> Switch3/2, Abs3/1, Abs6/1
  m/s to mm/s5/1 -> push0_2/1
  Abs6/1 -> m/s to mm/s6/1
  m/s to mm/s6/1 -> pull_2/1
  push0_2/1 -> Gain/1
  Gain1/1 -> Product1/2  "wheel_travel_velocity"
  Roll_Angle-MR_frontright/1 -> Product1/1  "MR"
  m/s to mm/s4/1 -> pull_1/1
  Abs2/1 -> m/s to mm/s4/1
  m/s to mm/s1/1 -> push0_1/1
  Product2/1 -> Abs1/1, Switch2/2, Abs2/1
  Abs1/1 -> m/s to mm/s1/1
  Switch1/1 -> Add1/1
  Abs5/1 -> m/s to mm/s2/1
  Gain6/1 -> Product4/2  "wheel_travel_velocity"
  Abs4/1 -> m/s to mm/s3/1
  Roll_Angle-MR_rearleft/1 -> Product4/1  "MR"
  Product4/1 -> Switch1/2, Abs5/1, Abs4/1
  m/s to mm/s2/1 -> push0_/1
  m/s to mm/s3/1 -> pull_/1
  Gain5/1 -> Product2/2  "wheel_travel_velocity"
  "rear "/1 -> Gain6/1, Gain2/1, Roll_Angle-MR_rearright/1, Roll_Angle-MR_rearleft/1
  "front "/1 -> Gain5/1, Roll_Angle-MR_frontright/1, Gain1/1, Roll_Angle-MR_frontleft/1
  Roll_Angle-MR_frontleft/1 -> Product2/1  "MR"
  Add1/1 -> Rear_Axle_force [N]/1
  Gain/1 -> Switch3/1
  Gain3/1 -> Switch3/3
  push0_3/1 -> Switch4/1
  Gain4/1 -> Switch1/1
  Gain7/1 -> Switch1/3

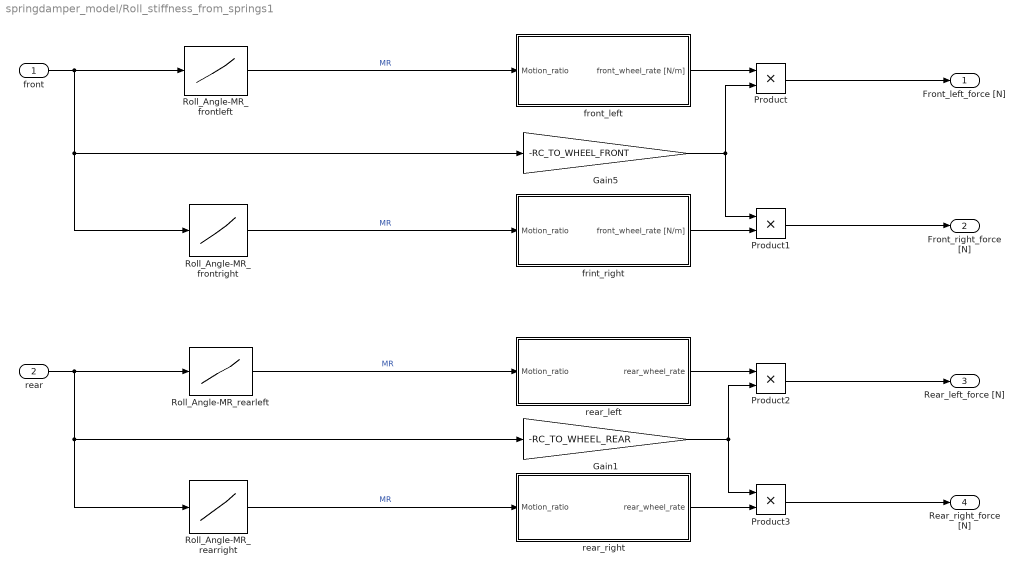
== system springdamper_model/Roll_stiffness_from_springs1 ==
  front : Inport
  rear : Inport  Port=2
  Gain1 : Gain  Gain=-RC_TO_WHEEL_REAR
  Gain5 : Gain  Gain=-RC_TO_WHEEL_FRONT
  Product{,1..3} (4 alike) : Product
  Roll_Angle-MR_frontleft : Lookup_n-D  NumberOfTableDimensions=1  BreakpointsForDimension1=[-0.02618 -0.02356 -0.02094 -0.01833 -0.01571 -0.01309 -0.01047 -0.00785 -0.00524 -0.00262 0.00000 0.00262 0.00524 0.00785 0.01047 0.01309 0.01571 0.01833 0.02094 0.02356 0.02618]  Table=[1.013 1.023 1.032 1.042 1.052 1.062 1.073 1.083 1.093 1.104 1.114 1.125 1.136 1.147 1.158 1.169 1.181 1.192 1.204 1.215 1.227]  InternalRulePriority=Speed  RndMeth=Simplest  InputSameDT=on
  Roll_Angle-MR_frontright : Lookup_n-D  NumberOfTableDimensions=1  BreakpointsForDimension1=[-0.02618 -0.02356 -0.02094 -0.01833 -0.01571 -0.01309 -0.01047 -0.00785 -0.00524 -0.00262 0.00000 0.00262 0.00524 0.00785 0.01047 0.01309 0.01571 0.01833 0.02094 0.02356 0.02618]  Table=[1.227 1.215 1.204 1.192 1.181 1.169 1.158 1.147 1.136 1.125 1.115 1.104 1.093 1.083 1.073 1.062 1.052 1.042 1.032 1.023 1.013]  InternalRulePriority=Speed  RndMeth=Simplest  InputSameDT=on
  Roll_Angle-MR_rearleft : Lookup_n-D  NumberOfTableDimensions=1  BreakpointsForDimension1=[-0.02618 -0.02356 -0.02094 -0.01833 -0.01571 -0.01309 -0.01047 -0.00785 -0.00524 -0.00262 0.00000 0.00262 0.00524 0.00785 0.01047 0.01309 0.01571 0.01833 0.02094 0.02356 0.02618]  Table=[0.945 0.953 0.962 0.971 0.980 0.990 0.999 1.009 1.019 1.029 1.039 1.049 1.059 1.070 1.080 1.091 1.102 1.113 1.124 1.135 1.147]  InternalRulePriority=Speed  RndMeth=Simplest  InputSameDT=on
  Roll_Angle-MR_rearright : Lookup_n-D  NumberOfTableDimensions=1  BreakpointsForDimension1=[-0.02618 -0.02356 -0.02094 -0.01833 -0.01571 -0.01309 -0.01047 -0.00785 -0.00524 -0.00262 0.00000 0.00262 0.00524 0.00785 0.01047 0.01309 0.01571 0.01833 0.02094 0.02356 0.02618]  Table=[1.147 1.135 1.124 1.113 1.102 1.091 1.080 1.070 1.059 1.049 1.039 1.029 1.019 1.009 0.999 0.990 0.980 0.971 0.962 0.953 0.945]  InternalRulePriority=Speed  RndMeth=Simplest  InputSameDT=on
  frint_right : Subsystem
  front_left : Subsystem
  rear_left : Subsystem
  rear_right : Subsystem
  Front_left_force [N] : Outport
  Front_right_force [N] : Outport  Port=2
  Rear_left_force [N] : Outport  Port=3
  Rear_right_force [N] : Outport  Port=4
  wires:
  rear_left/1(rear_wheel_rate) -> Product2/1
  front_left/1(front_wheel_rate [N/m]) -> Product/1
  front/1 -> Gain5/1, Roll_Angle-MR_frontright/1, Roll_Angle-MR_frontleft/1
  rear/1 -> Roll_Angle-MR_rearleft/1, Gain1/1, Roll_Angle-MR_rearright/1
  Roll_Angle-MR_rearleft/1 -> rear_left/1(Motion_ratio)  "MR"
  Roll_Angle-MR_frontleft/1 -> front_left/1(Motion_ratio)  "MR"
  Roll_Angle-MR_frontright/1 -> frint_right/1(Motion_ratio)  "MR"
  Roll_Angle-MR_rearright/1 -> rear_right/1(Motion_ratio)  "MR"
  frint_right/1(front_wheel_rate [N/m]) -> Product1/2
  rear_right/1(rear_wheel_rate) -> Product3/2
  Gain5/1 -> Product1/1, Product/2
  Product/1 -> Front_left_force [N]/1
  Gain1/1 -> Product3/1, Product2/2
  Product2/1 -> Rear_left_force [N]/1
  Product1/1 -> Front_right_force [N]/1
  Product3/1 -> Rear_right_force [N]/1

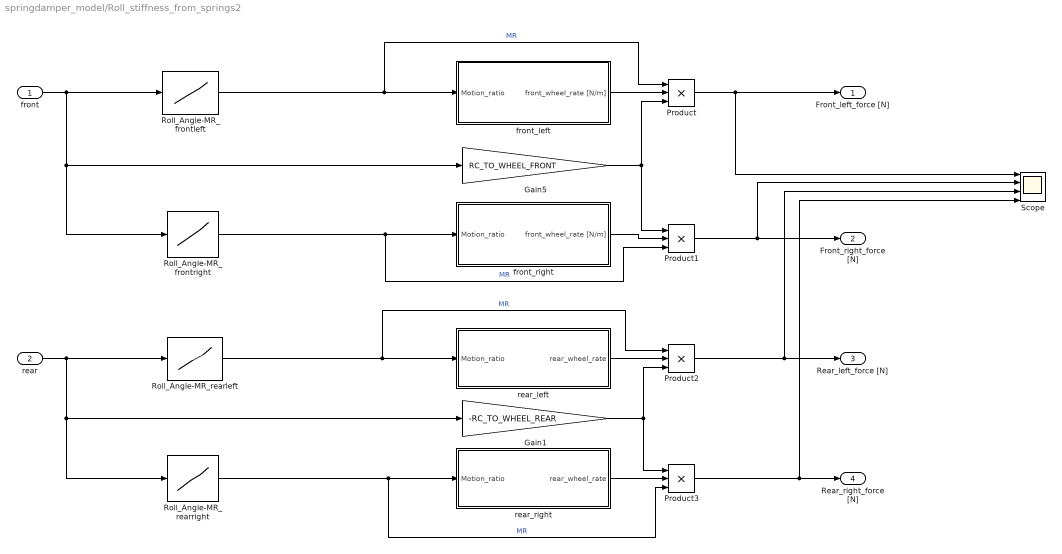
== system springdamper_model/Roll_stiffness_from_springs2 ==
  front : Inport
  rear : Inport  Port=2
  Gain1 : Gain  Gain=-RC_TO_WHEEL_REAR
  Gain5 : Gain  Gain=RC_TO_WHEEL_FRONT
  Product{,1..3} (4 alike) : Product  Inputs=3
  Roll_Angle-MR_frontleft : Lookup_n-D  NumberOfTableDimensions=1  BreakpointsForDimension1=[-0.02618 -0.02356 -0.02094 -0.01833 -0.01571 -0.01309 -0.01047 -0.00785 -0.00524 -0.00262 0.00000 0.00262 0.00524 0.00785 0.01047 0.01309 0.01571 0.01833 0.02094 0.02356 0.02618]  Table=[1.013 1.023 1.032 1.042 1.052 1.062 1.073 1.083 1.093 1.104 1.114 1.125 1.136 1.147 1.158 1.169 1.181 1.192 1.204 1.215 1.227]  InternalRulePriority=Speed  RndMeth=Simplest  InputSameDT=on
  Roll_Angle-MR_frontright : Lookup_n-D  NumberOfTableDimensions=1  BreakpointsForDimension1=[-0.02618 -0.02356 -0.02094 -0.01833 -0.01571 -0.01309 -0.01047 -0.00785 -0.00524 -0.00262 0.00000 0.00262 0.00524 0.00785 0.01047 0.01309 0.01571 0.01833 0.02094 0.02356 0.02618]  Table=[1.227 1.215 1.204 1.192 1.181 1.169 1.158 1.147 1.136 1.125 1.115 1.104 1.093 1.083 1.073 1.062 1.052 1.042 1.032 1.023 1.013]  InternalRulePriority=Speed  RndMeth=Simplest  InputSameDT=on
  Roll_Angle-MR_rearleft : Lookup_n-D  NumberOfTableDimensions=1  BreakpointsForDimension1=[-0.02618 -0.02356 -0.02094 -0.01833 -0.01571 -0.01309 -0.01047 -0.00785 -0.00524 -0.00262 0.00000 0.00262 0.00524 0.00785 0.01047 0.01309 0.01571 0.01833 0.02094 0.02356 0.02618]  Table=[0.945 0.953 0.962 0.971 0.980 0.990 0.999 1.009 1.019 1.029 1.039 1.049 1.059 1.070 1.080 1.091 1.102 1.113 1.124 1.135 1.147]  InternalRulePriority=Speed  RndMeth=Simplest  InputSameDT=on
  Roll_Angle-MR_rearright : Lookup_n-D  NumberOfTableDimensions=1  BreakpointsForDimension1=[-0.02618 -0.02356 -0.02094 -0.01833 -0.01571 -0.01309 -0.01047 -0.00785 -0.00524 -0.00262 0.00000 0.00262 0.00524 0.00785 0.01047 0.01309 0.01571 0.01833 0.02094 0.02356 0.02618]  Table=[1.147 1.135 1.124 1.113 1.102 1.091 1.080 1.070 1.059 1.049 1.039 1.029 1.019 1.009 0.999 0.990 0.980 0.971 0.962 0.953 0.945]  InternalRulePriority=Speed  RndMeth=Simplest  InputSameDT=on
  Scope : Scope  NumInputPorts=4
  front_left : Subsystem
  front_right : Subsystem
  rear_left : Subsystem
  rear_right : Subsystem
  Front_left_force [N] : Outport
  Front_right_force [N] : Outport  Port=2
  Rear_left_force [N] : Outport  Port=3
  Rear_right_force [N] : Outport  Port=4
  wires:
  Product3/1 -> Scope/4, Rear_right_force [N]/1
  Product1/1 -> Scope/2, Front_right_force [N]/1
  Product2/1 -> Scope/3, Rear_left_force [N]/1
  Gain1/1 -> Product2/3, Product3/1
  Product/1 -> Scope/1, Front_left_force [N]/1
  Gain5/1 -> Product/3, Product1/1
  rear_right/1(rear_wheel_rate) -> Product3/2
  front_right/1(front_wheel_rate [N/m]) -> Product1/2
  Roll_Angle-MR_rearright/1 -> Product3/3, rear_right/1(Motion_ratio)  "MR"
  Roll_Angle-MR_frontright/1 -> Product1/3, front_right/1(Motion_ratio)  "MR"
  Roll_Angle-MR_frontleft/1 -> Product/1, front_left/1(Motion_ratio)  "MR"
  Roll_Angle-MR_rearleft/1 -> Product2/1, rear_left/1(Motion_ratio)  "MR"
  rear/1 -> Roll_Angle-MR_rearright/1, Gain1/1, Roll_Angle-MR_rearleft/1
  front/1 -> Roll_Angle-MR_frontleft/1, Roll_Angle-MR_frontright/1, Gain5/1
  front_left/1(front_wheel_rate [N/m]) -> Product/2
  rear_left/1(rear_wheel_rate) -> Product2/2

== system springdamper_model/Signal Builder1 ==
  Demux : Demux  Tag=STV Demux  Outputs=2
      settings: DisplayOption=none
  FromWs : FromWorkspace  Tag=STV FromWs  VariableName=tuvar
      SigBuilderData=|
      | common.afterFinalStr = 'Extrapolate'
      | common.sampleTime = 0
      | dataSet.timeRange = [0 4]
      | dataSet.name = 'Group 1'
      | sbobj.Groups.Name = 'Group 1'
      | sbobj.Groups.Signals(1).Name = 'Signal 1'
      | sbobj.Groups.Signals(1).XData = [0 1 1 1.01 1.01 4]
      | sbobj.Groups.Signals(1).YData = [0 0 0.01 0.01 0 0]
      | sbobj.Groups.Signals(2).Name = 'Signal 2'
      | sbobj.Groups.Signals(2).XData = [0 1 1 4]
      | sbobj.Groups.Signals(2).YData = [0 0 0.01 0.01]
      | sbobj.Groups.TimeRange = [0 4]
  Signal 1 : Outport  Tag=STV Outport
  Signal 2 : Outport  Tag=STV Outport  Port=2
  wires:
  FromWs/1 -> Demux/1
  Demux/1 -> Signal 1/1
  Demux/2 -> Signal 2/1

== system springdamper_model/Signal Builder2 ==
  Demux : Demux  Tag=STV Demux  Outputs=2
      settings: DisplayOption=none
  FromWs : FromWorkspace  Tag=STV FromWs  VariableName=tuvar
      SigBuilderData=|
      | common.afterFinalStr = 'Extrapolate'
      | common.sampleTime = 0
      | dataSet.timeRange = [0 5]
      | dataSet.name = 'Group 1'
      | sbobj.Groups.Name = 'Group 1'
      | sbobj.Groups.Signals(1).Name = 'Signal 1'
      | sbobj.Groups.Signals(1).XData = [0 1 1 1.01 1.01 5]
      | sbobj.Groups.Signals(1).YData = [0 0 9.81 9.81 0 0]
      | sbobj.Groups.Signals(2).Name = 'Signal 2'
      | sbobj.Groups.Signals(2).XData = [0 1 1 5]
      | sbobj.Groups.Signals(2).YData = [0 0 9.81 9.81]
      | sbobj.Groups.TimeRange = [0 5]
  Signal 1 : Outport  Tag=STV Outport
  Signal 2 : Outport  Tag=STV Outport  Port=2
  wires:
  FromWs/1 -> Demux/1
  Demux/1 -> Signal 1/1
  Demux/2 -> Signal 2/1

== system springdamper_model/Signal Builder3 ==
  Demux : Demux  Tag=STV Demux  Outputs=2
      settings: DisplayOption=none
  FromWs : FromWorkspace  Tag=STV FromWs  VariableName=tuvar
      SigBuilderData=|
      | common.afterFinalStr = 'Extrapolate'
      | common.sampleTime = 0
      | dataSet.timeRange = [0 5]
      | dataSet.name = 'Group 1'
      | sbobj.Groups.Name = 'Group 1'
      | sbobj.Groups.Signals(1).Name = 'Signal 1'
      | sbobj.Groups.Signals(1).XData = [0 1 1 1.01 1.01 5]
      | sbobj.Groups.Signals(1).YData = [0 0 9.81 9.81 0 0]
      | sbobj.Groups.Signals(2).Name = 'Signal 2'
      | sbobj.Groups.Signals(2).XData = [0 1 1 5]
      | sbobj.Groups.Signals(2).YData = [0 0 9.81 9.81]
      | sbobj.Groups.TimeRange = [0 5]
  Signal 1 : Outport  Tag=STV Outport
  Signal 2 : Outport  Tag=STV Outport  Port=2
  wires:
  Demux/2 -> Signal 2/1
  Demux/1 -> Signal 1/1
  FromWs/1 -> Demux/1

== system springdamper_model/Signal Builder4 ==
  Demux : Demux  Tag=STV Demux  Outputs=2
      settings: DisplayOption=none
  FromWs : FromWorkspace  Tag=STV FromWs  VariableName=tuvar
      SigBuilderData=|
      | common.afterFinalStr = 'Extrapolate'
      | common.sampleTime = 0
      | dataSet.timeRange = [0 4]
      | dataSet.name = 'Group 1'
      | sbobj.Groups.Name = 'Group 1'
      | sbobj.Groups.Signals(1).Name = 'Signal 1'
      | sbobj.Groups.Signals(1).XData = [0 1 1 1.01 1.01 4]
      | sbobj.Groups.Signals(1).YData = [0 0 0.01 0.01 0 0]
      | sbobj.Groups.Signals(2).Name = 'Signal 2'
      | sbobj.Groups.Signals(2).XData = [0 1 1 4]
      | sbobj.Groups.Signals(2).YData = [0 0 0.01 0.01]
      | sbobj.Groups.TimeRange = [0 4]
  Signal 1 : Outport  Tag=STV Outport
  Signal 2 : Outport  Tag=STV Outport  Port=2
  wires:
  Demux/2 -> Signal 2/1
  Demux/1 -> Signal 1/1
  FromWs/1 -> Demux/1

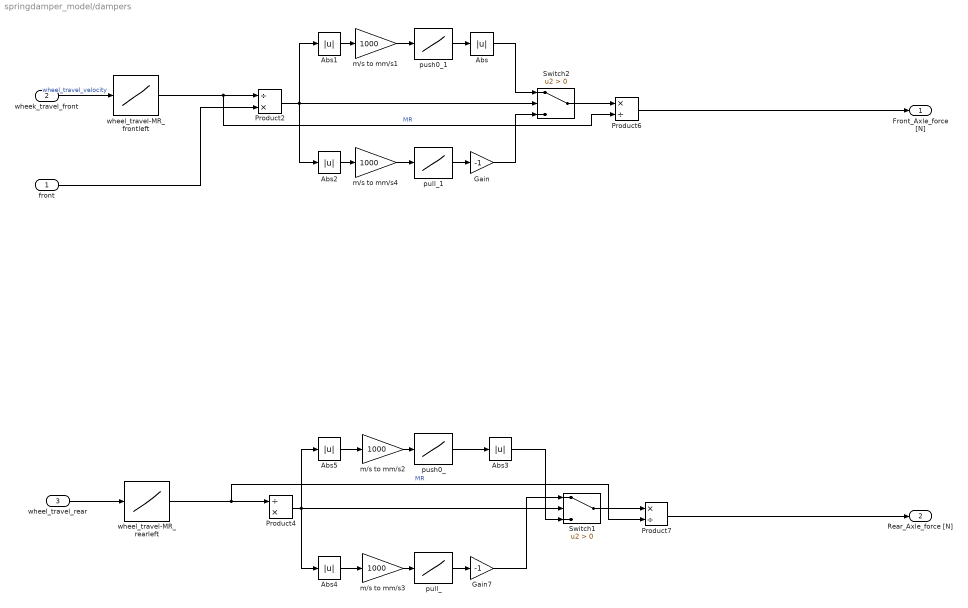
== system springdamper_model/dampers ==
  "front " : Inport
  wheek_travel_front : Inport  Port=2
  "wheel_travel_rear " : Inport  Port=3
  Abs{,1..5} (6 alike) : Abs
  Gain : Gain  Gain=-1
  Gain7 : Gain  Gain=-1
  Product2 : Product  Inputs=/*
  Product4 : Product  Inputs=/*
  Product6 : Product  Inputs=*/
  Product7 : Product  Inputs=*/
  Switch1 : Switch  Criteria=u2 > Threshold
  Switch2 : Switch  Criteria=u2 > Threshold
  m/s to mm/s{1..4} (4 alike) : Gain  Gain=1000
  pull_ : Lookup_n-D  NumberOfTableDimensions=1  BreakpointsForDimension1=vel  Table=pull  InternalRulePriority=Speed  RndMeth=Simplest  InputSameDT=on
  pull_1 : Lookup_n-D  NumberOfTableDimensions=1  BreakpointsForDimension1=vel  Table=pull  InternalRulePriority=Speed  RndMeth=Simplest  InputSameDT=on
  push0_ : Lookup_n-D  NumberOfTableDimensions=1  BreakpointsForDimension1=vel  Table=push  InternalRulePriority=Speed  RndMeth=Simplest  InputSameDT=on
  push0_1 : Lookup_n-D  NumberOfTableDimensions=1  BreakpointsForDimension1=vel  Table=push  InternalRulePriority=Speed  RndMeth=Simplest  InputSameDT=on
  wheel_travel-MR_frontleft : Lookup_n-D  NumberOfTableDimensions=1  BreakpointsForDimension1=[-25.0 -22.5 -20.0 -17.5 -15.0 -12.5 -10.0 -7.5 -5.0 -2.5 0.0 2.5 5.0 7.5 10.0 12.5 15.0 17.5 20.0 22.5 25.0]  Table=[1.2992 1.2797 1.2606 1.2418 1.2232 1.2050 1.1870 1.1662 1.1487 1.1316 1.1147 1.0980 1.0816 1.0654 1.0495 1.0339 1.0186 1.0035 0.9888 0.9744 0.9604]  InternalRulePriority=Speed  RndMeth=Simplest  InputSameDT=on
  wheel_travel-MR_rearleft : Lookup_n-D  NumberOfTableDimensions=1  BreakpointsForDimension1=[-25.0 -22.5 -20.0 -17.5 -15.0 -12.5 -10.0 -7.5 -5.0 -2.5 0.0 2.5 5.0 7.5 10.0 12.5 15.0 17.5 20.0 22.5 25.0]  Table=|  InternalRulePriority=Speed  RndMeth=Simplest  InputSameDT=on
      | [1.2145 1.1957 1.1771 1.1589 1.1410 1.1233 1.1059 1.0887 1.0719 1.0553 1.0390 1.0230 1.0073 0.9920 0.9770 0.9625 0.9484 0.9348 0.9217 0.9093 0.8977
      | ]
  Front_Axle_force [N] : Outport
  Rear_Axle_force [N] : Outport  Port=2
  wires:
  Gain7/1 -> Switch1/1
  Abs3/1 -> Switch1/3
  Product6/1 -> Front_Axle_force [N]/1
  m/s to mm/s4/1 -> pull_1/1
  Abs2/1 -> m/s to mm/s4/1
  pull_1/1 -> Gain/1
  m/s to mm/s1/1 -> push0_1/1
  Product2/1 -> Abs1/1, Switch2/2, Abs2/1
  Abs1/1 -> m/s to mm/s1/1
  push0_/1 -> Abs3/1
  pull_/1 -> Gain7/1
  Abs5/1 -> m/s to mm/s2/1
  Abs4/1 -> m/s to mm/s3/1
  Switch1/1 -> Product7/1
  wheel_travel-MR_rearleft/1 -> Product4/1, Product7/2  "MR"
  Product4/1 -> Switch1/2, Abs5/1, Abs4/1
  m/s to mm/s2/1 -> push0_/1
  m/s to mm/s3/1 -> pull_/1
  "wheel_travel_rear "/1 -> wheel_travel-MR_rearleft/1
  "front "/1 -> Product2/2
  wheel_travel-MR_frontleft/1 -> Product2/1, Product6/2  "MR"
  Product7/1 -> Rear_Axle_force [N]/1
  Switch2/1 -> Product6/1
  wheek_travel_front/1 -> wheel_travel-MR_frontleft/1  "wheel_travel_velocity"
  push0_1/1 -> Abs/1
  Gain/1 -> Switch2/3
  Abs/1 -> Switch2/1

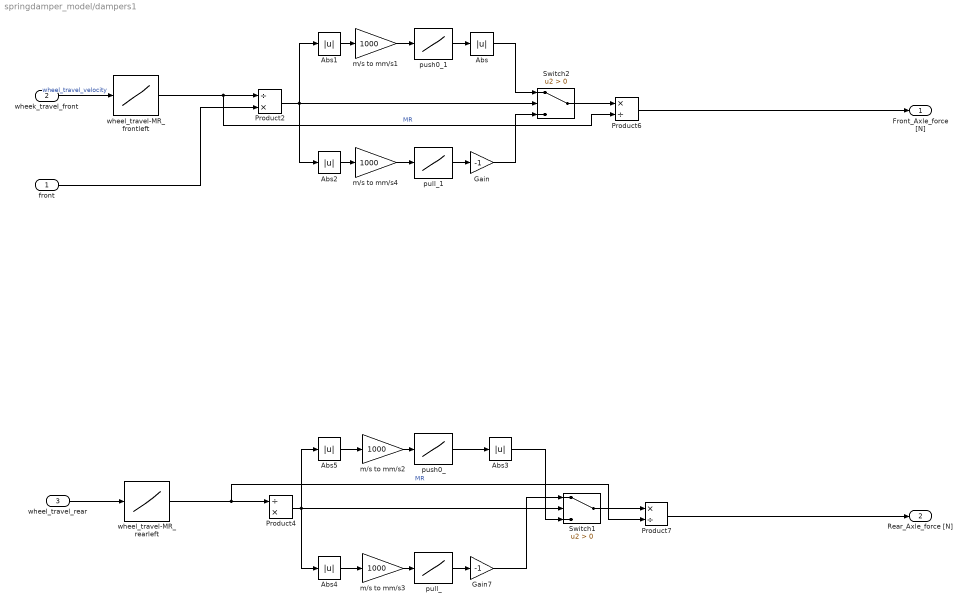
== system springdamper_model/dampers1 ==
  "front " : Inport
  wheek_travel_front : Inport  Port=2
  "wheel_travel_rear " : Inport  Port=3
  Abs{,1..5} (6 alike) : Abs
  Gain : Gain  Gain=-1
  Gain7 : Gain  Gain=-1
  Product2 : Product  Inputs=/*
  Product4 : Product  Inputs=/*
  Product6 : Product  Inputs=*/
  Product7 : Product  Inputs=*/
  Switch1 : Switch  Criteria=u2 > Threshold
  Switch2 : Switch  Criteria=u2 > Threshold
  m/s to mm/s{1..4} (4 alike) : Gain  Gain=1000
  pull_ : Lookup_n-D  NumberOfTableDimensions=1  BreakpointsForDimension1=vel  Table=pull  InternalRulePriority=Speed  RndMeth=Simplest  InputSameDT=on
  pull_1 : Lookup_n-D  NumberOfTableDimensions=1  BreakpointsForDimension1=vel  Table=pull  InternalRulePriority=Speed  RndMeth=Simplest  InputSameDT=on
  push0_ : Lookup_n-D  NumberOfTableDimensions=1  BreakpointsForDimension1=vel  Table=push  InternalRulePriority=Speed  RndMeth=Simplest  InputSameDT=on
  push0_1 : Lookup_n-D  NumberOfTableDimensions=1  BreakpointsForDimension1=vel  Table=push  InternalRulePriority=Speed  RndMeth=Simplest  InputSameDT=on
  wheel_travel-MR_frontleft : Lookup_n-D  NumberOfTableDimensions=1  BreakpointsForDimension1=[-25.0 -22.5 -20.0 -17.5 -15.0 -12.5 -10.0 -7.5 -5.0 -2.5 0.0 2.5 5.0 7.5 10.0 12.5 15.0 17.5 20.0 22.5 25.0]  Table=[1.2992 1.2797 1.2606 1.2418 1.2232 1.2050 1.1870 1.1662 1.1487 1.1316 1.1147 1.0980 1.0816 1.0654 1.0495 1.0339 1.0186 1.0035 0.9888 0.9744 0.9604]  InternalRulePriority=Speed  RndMeth=Simplest  InputSameDT=on
  wheel_travel-MR_rearleft : Lookup_n-D  NumberOfTableDimensions=1  BreakpointsForDimension1=[-25.0 -22.5 -20.0 -17.5 -15.0 -12.5 -10.0 -7.5 -5.0 -2.5 0.0 2.5 5.0 7.5 10.0 12.5 15.0 17.5 20.0 22.5 25.0]  Table=|  InternalRulePriority=Speed  RndMeth=Simplest  InputSameDT=on
      | [1.2145 1.1957 1.1771 1.1589 1.1410 1.1233 1.1059 1.0887 1.0719 1.0553 1.0390 1.0230 1.0073 0.9920 0.9770 0.9625 0.9484 0.9348 0.9217 0.9093 0.8977
      | ]
  Front_Axle_force [N] : Outport
  Rear_Axle_force [N] : Outport  Port=2
  wires:
  Gain7/1 -> Switch1/1
  Abs3/1 -> Switch1/3
  Product6/1 -> Front_Axle_force [N]/1
  m/s to mm/s4/1 -> pull_1/1
  Abs2/1 -> m/s to mm/s4/1
  pull_1/1 -> Gain/1
  m/s to mm/s1/1 -> push0_1/1
  Product2/1 -> Abs1/1, Switch2/2, Abs2/1
  Abs1/1 -> m/s to mm/s1/1
  push0_/1 -> Abs3/1
  pull_/1 -> Gain7/1
  Abs5/1 -> m/s to mm/s2/1
  Abs4/1 -> m/s to mm/s3/1
  Switch1/1 -> Product7/1
  wheel_travel-MR_rearleft/1 -> Product4/1, Product7/2  "MR"
  Product4/1 -> Switch1/2, Abs5/1, Abs4/1
  m/s to mm/s2/1 -> push0_/1
  m/s to mm/s3/1 -> pull_/1
  "wheel_travel_rear "/1 -> wheel_travel-MR_rearleft/1
  "front "/1 -> Product2/2
  wheel_travel-MR_frontleft/1 -> Product2/1, Product6/2  "MR"
  Product7/1 -> Rear_Axle_force [N]/1
  Switch2/1 -> Product6/1
  wheek_travel_front/1 -> wheel_travel-MR_frontleft/1  "wheel_travel_velocity"
  push0_1/1 -> Abs/1
  Gain/1 -> Switch2/3
  Abs/1 -> Switch2/1

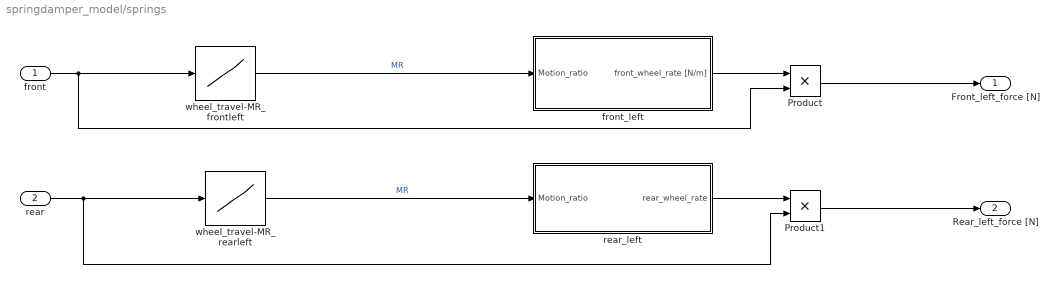
== system springdamper_model/springs ==
  front : Inport
  rear : Inport  Port=2
  Product : Product
  Product1 : Product
  front_left : Subsystem
  rear_left : Subsystem
  wheel_travel-MR_frontleft : Lookup_n-D  NumberOfTableDimensions=1  BreakpointsForDimension1=[-25.0 -22.5 -20.0 -17.5 -15.0 -12.5 -10.0 -7.5 -5.0 -2.5 0.0 2.5 5.0 7.5 10.0 12.5 15.0 17.5 20.0 22.5 25.0]  Table=[1.2992 1.2797 1.2606 1.2418 1.2232 1.2050 1.1870 1.1662 1.1487 1.1316 1.1147 1.0980 1.0816 1.0654 1.0495 1.0339 1.0186 1.0035 0.9888 0.9744 0.9604]  InternalRulePriority=Speed  RndMeth=Simplest  InputSameDT=on
  wheel_travel-MR_rearleft : Lookup_n-D  NumberOfTableDimensions=1  BreakpointsForDimension1=[-25.0 -22.5 -20.0 -17.5 -15.0 -12.5 -10.0 -7.5 -5.0 -2.5 0.0 2.5 5.0 7.5 10.0 12.5 15.0 17.5 20.0 22.5 25.0]  Table=|  InternalRulePriority=Speed  RndMeth=Simplest  InputSameDT=on
      | [1.2145 1.1957 1.1771 1.1589 1.1410 1.1233 1.1059 1.0887 1.0719 1.0553 1.0390 1.0230 1.0073 0.9920 0.9770 0.9625 0.9484 0.9348 0.9217 0.9093 0.8977
      | ]
  Front_left_force [N] : Outport
  Rear_left_force [N] : Outport  Port=2
  wires:
  rear_left/1(rear_wheel_rate) -> Product1/1
  front_left/1(front_wheel_rate [N/m]) -> Product/1
  wheel_travel-MR_frontleft/1 -> front_left/1(Motion_ratio)  "MR"
  wheel_travel-MR_rearleft/1 -> rear_left/1(Motion_ratio)  "MR"
  rear/1 -> Product1/2, wheel_travel-MR_rearleft/1
  front/1 -> Product/2, wheel_travel-MR_frontleft/1
  Product/1 -> Front_left_force [N]/1
  Product1/1 -> Rear_left_force [N]/1

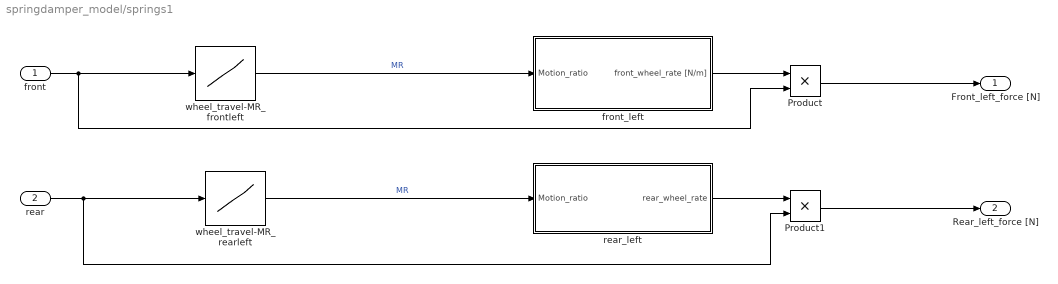
== system springdamper_model/springs1 ==
  front : Inport
  rear : Inport  Port=2
  Product : Product
  Product1 : Product
  front_left : Subsystem
  rear_left : Subsystem
  wheel_travel-MR_frontleft : Lookup_n-D  NumberOfTableDimensions=1  BreakpointsForDimension1=[-25.0 -22.5 -20.0 -17.5 -15.0 -12.5 -10.0 -7.5 -5.0 -2.5 0.0 2.5 5.0 7.5 10.0 12.5 15.0 17.5 20.0 22.5 25.0]  Table=[1.2992 1.2797 1.2606 1.2418 1.2232 1.2050 1.1870 1.1662 1.1487 1.1316 1.1147 1.0980 1.0816 1.0654 1.0495 1.0339 1.0186 1.0035 0.9888 0.9744 0.9604]  InternalRulePriority=Speed  RndMeth=Simplest  InputSameDT=on
  wheel_travel-MR_rearleft : Lookup_n-D  NumberOfTableDimensions=1  BreakpointsForDimension1=[-25.0 -22.5 -20.0 -17.5 -15.0 -12.5 -10.0 -7.5 -5.0 -2.5 0.0 2.5 5.0 7.5 10.0 12.5 15.0 17.5 20.0 22.5 25.0]  Table=|  InternalRulePriority=Speed  RndMeth=Simplest  InputSameDT=on
      | [1.2145 1.1957 1.1771 1.1589 1.1410 1.1233 1.1059 1.0887 1.0719 1.0553 1.0390 1.0230 1.0073 0.9920 0.9770 0.9625 0.9484 0.9348 0.9217 0.9093 0.8977
      | ]
  Front_left_force [N] : Outport
  Rear_left_force [N] : Outport  Port=2
  wires:
  rear_left/1(rear_wheel_rate) -> Product1/1
  front_left/1(front_wheel_rate [N/m]) -> Product/1
  wheel_travel-MR_frontleft/1 -> front_left/1(Motion_ratio)  "MR"
  wheel_travel-MR_rearleft/1 -> rear_left/1(Motion_ratio)  "MR"
  rear/1 -> Product1/2, wheel_travel-MR_rearleft/1
  front/1 -> Product/2, wheel_travel-MR_frontleft/1
  Product/1 -> Front_left_force [N]/1
  Product1/1 -> Rear_left_force [N]/1

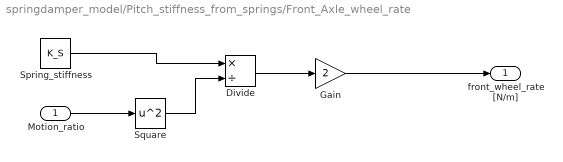
== system springdamper_model/Pitch_stiffness_from_springs/Front_Axle_wheel_rate ==
  Motion_ratio : Inport
  Divide : Product  Inputs=*/
  Gain : Gain  Gain=2
  Spring_stiffness : Constant  Value=K_S
  Square : Math  Operator=square  SaturateOnIntegerOverflow=on
  front_wheel_rate [N/m] : Outport
  wires:
  Motion_ratio/1 -> Square/1
  Divide/1 -> Gain/1
  Square/1 -> Divide/2
  Gain/1 -> front_wheel_rate [N/m]/1
  Spring_stiffness/1 -> Divide/1

== system springdamper_model/Pitch_stiffness_from_springs/Rear_Axle_wheel_rate ==
  Motion_ratio : Inport
  Divide1 : Product  Inputs=*/
  Gain1 : Gain  Gain=2
  Spring_stiffness1 : Constant  Value=K_S
  Square1 : Math  Operator=square  SaturateOnIntegerOverflow=on
  rear_wheel_rate : Outport
  wires:
  Gain1/1 -> rear_wheel_rate/1
  Square1/1 -> Divide1/2
  Spring_stiffness1/1 -> Divide1/1
  Divide1/1 -> Gain1/1
  Motion_ratio/1 -> Square1/1

== system springdamper_model/Roll_stiffness_from_springs1/frint_right ==
  Motion_ratio : Inport
  Divide : Product  Inputs=*/
  Spring_stiffness : Constant  Value=K_S
  Square : Math  Operator=square  SaturateOnIntegerOverflow=on
  front_wheel_rate [N/m] : Outport
  wires:
  Spring_stiffness/1 -> Divide/1
  Divide/1 -> front_wheel_rate [N/m]/1
  Motion_ratio/1 -> Square/1
  Square/1 -> Divide/2

== system springdamper_model/Roll_stiffness_from_springs1/front_left ==
  Motion_ratio : Inport
  Divide : Product  Inputs=*/
  Spring_stiffness : Constant  Value=K_S
  Square : Math  Operator=square  SaturateOnIntegerOverflow=on
  front_wheel_rate [N/m] : Outport
  wires:
  Divide/1 -> front_wheel_rate [N/m]/1
  Spring_stiffness/1 -> Divide/1
  Motion_ratio/1 -> Square/1
  Square/1 -> Divide/2

== system springdamper_model/Roll_stiffness_from_springs1/rear_left ==
  Motion_ratio : Inport
  Divide1 : Product  Inputs=*/
  Spring_stiffness1 : Constant  Value=K_S
  Square1 : Math  Operator=square  SaturateOnIntegerOverflow=on
  rear_wheel_rate : Outport
  wires:
  Divide1/1 -> rear_wheel_rate/1
  Spring_stiffness1/1 -> Divide1/1
  Motion_ratio/1 -> Square1/1
  Square1/1 -> Divide1/2

== system springdamper_model/Roll_stiffness_from_springs1/rear_right ==
  Motion_ratio : Inport
  Divide1 : Product  Inputs=*/
  Spring_stiffness1 : Constant  Value=K_S
  Square1 : Math  Operator=square  SaturateOnIntegerOverflow=on
  rear_wheel_rate : Outport
  wires:
  Spring_stiffness1/1 -> Divide1/1
  Motion_ratio/1 -> Square1/1
  Divide1/1 -> rear_wheel_rate/1
  Square1/1 -> Divide1/2

== system springdamper_model/Roll_stiffness_from_springs2/front_left ==
  Motion_ratio : Inport
  Divide : Product  Inputs=*/
  Spring_stiffness : Constant  Value=K_S
  Square : Math  Operator=square  SaturateOnIntegerOverflow=on
  front_wheel_rate [N/m] : Outport
  wires:
  Spring_stiffness/1 -> Divide/1
  Divide/1 -> front_wheel_rate [N/m]/1
  Square/1 -> Divide/2
  Motion_ratio/1 -> Square/1

== system springdamper_model/Roll_stiffness_from_springs2/front_right ==
  Motion_ratio : Inport
  Divide : Product  Inputs=*/
  Spring_stiffness : Constant  Value=K_S
  Square : Math  Operator=square  SaturateOnIntegerOverflow=on
  front_wheel_rate [N/m] : Outport
  wires:
  Motion_ratio/1 -> Square/1
  Square/1 -> Divide/2
  Divide/1 -> front_wheel_rate [N/m]/1
  Spring_stiffness/1 -> Divide/1
